simulink library "ConverterLibrary"  (R2026a)
settings: Solver=VariableStepAuto
undefined symbols (not defined in the file or in its folder): DiscIntNeverNeededParam, dspblkCoreblockFVToolHelper, gcbh, gridInverter
libraries: fl_lib x240, nesl_utility x221, ee_lib x208, slpidlib x28, eeGeneralControl x12, simulink x9, eeTransforms x4, simulink_extras x1, eePowerMeasurement x1
(part 11 of 30)

== system ConverterLibrary/Power Converter Plant/Soft-Switching Converters/LLC Converter/LLC Primary Inverter and Resonant Tank/LLC Simplified Model ==
  G : Inport
  Inverter : Subsystem
      settings: PortSchema="{\"entries\":[{\"content\":{\"sides\":[{\"content\":{\"connectorIds\":[\"LConn1\",\"LConn2\"]},\"type\":\"ConnectorPlacement.EquallySpacedRectSide\",\"uuid\":\"5f98eff0-54e4-47a8-aeeb-0279cba14f26\"},{\"content\":{\"connectorIds\":[\"RConn1\",\"RConn2\"],\"side\":\"RIGHT\"},\"type\":\"ConnectorPlacement.EquallySpacedRectSide\",\"uuid\":\"71acbbb6-1fc8-426c-b389-5d494eb18bfd\"},{\"content\":{\"connectorIds\":[\"In1\",\"Out1\"],\"side\":\"TOP\"},\"type\":\"ConnectorPlacement.EquallySpacedRectSide\",\"uuid\":\"dc77ee05-1f57-4323-bfda-b0076e2d1ee5\"}]},\"type\":\"ConnectorPlacement.EquallySpacedConnector\",\"uuid\":\"8d0b8c05-d5c5-4033-af60-ebdb639bdc40\"}],\"packageUris\":[\"http://schema.mathworks.com/mf0/Connector/R2020b\"],\"version\":\"1.0\"}"
  Resonant Tank : Subsystem
      settings: PortSchema="{\"entries\":[{\"content\":{\"sides\":[{\"content\":{\"connectorIds\":[\"LConn1\",\"LConn2\"]},\"type\":\"ConnectorPlacement.EquallySpacedRectSide\",\"uuid\":\"d505f362-3b8e-4dee-9b5b-731d75550efb\"},{\"content\":{\"connectorIds\":[\"RConn1\",\"RConn2\",\"RConn3\"],\"side\":\"RIGHT\"},\"type\":\"ConnectorPlacement.EquallySpacedRectSide\",\"uuid\":\"66ab4b84-9b7a-404b-b3f6-3ac1c371ea42\"},{\"content\":{\"connectorIds\":[\"Out1\"],\"side\":\"TOP\"},\"type\":\"ConnectorPlacement.EquallySpacedRectSide\",\"uuid\":\"00605859-d490-4a3b-aace-391362dfba7e\"}]},\"type\":\"ConnectorPlacement.EquallySpacedConnector\",\"uuid\":\"a210fe68-7181-499f-8e1c-ccfe71b42a4c\"}],\"packageUris\":[\"http://schema.mathworks.com/mf0/Connector/R2020b\"],\"version\":\"1.0\"}"
      mask Display: image('LLCTransformerIcon.png');
  Selector : Selector  InputPortWidth=4  IndexOptions=Index vector (dialog)  Indices=[1 2]  OutputSizes=1
  + : PMIOPort  Side=Left
  P2+ : PMIOPort  Port=2  Side=Right
  N2 : PMIOPort  Port=3  Side=Right
  - : PMIOPort  Port=4  Side=Left
  P2- : PMIOPort  Port=5  Side=Right
  measInv : Outport
  measTank : Outport  Port=2
  wires:
  Selector/1 -> Inverter/1(G)
  G/1 -> Selector/1
  Resonant Tank/1(meas) -> measTank/1  "ResonantTank"
  Inverter/1(meas) -> measInv/1  "Inverter"
  connections:
  Resonant Tank/RConn2 -- N2/RConn1
  +/RConn1 -- Inverter/LConn1
  Resonant Tank/RConn1 -- P2+/RConn1
  Resonant Tank/LConn2 -- Inverter/RConn2
  Resonant Tank/RConn3 -- P2-/RConn1
  Resonant Tank/LConn1 -- Inverter/RConn1
  -/RConn1 -- Inverter/LConn2

== system ConverterLibrary/Power Converter Plant/Soft-Switching Converters/LLC Converter/Rectifier/Iout ==
  Current Sensor : fl_lib/Electrical/Electrical Sensors/Current Sensor
  PS-Simulink Converter : nesl_utility/PS-Simulink Converter  PhysicalDomain=network_engine_domain  SubClassName=ps_output  LeftPortType=input  RightPortType=output  PseudoPeriodic=off  Frequencies=[]  VectorFormat=inherit  Unit=inherit  AffineConversion=off
  + : PMIOPort  Side=Left
  - : PMIOPort  Port=2  Side=Right
  I : Outport
  wires:
  PS-Simulink Converter/1 -> I/1
  connections:
  Current Sensor/RConn1 -- PS-Simulink Converter/LConn1
  +/RConn1 -- Current Sensor/LConn1
  Current Sensor/RConn2 -- -/RConn1

== system ConverterLibrary/Power Converter Plant/Soft-Switching Converters/LLC Converter/Rectifier/IoutRect ==
  Current Sensor : fl_lib/Electrical/Electrical Sensors/Current Sensor
  PS-Simulink Converter : nesl_utility/PS-Simulink Converter  PhysicalDomain=network_engine_domain  SubClassName=ps_output  LeftPortType=input  RightPortType=output  PseudoPeriodic=off  Frequencies=[]  VectorFormat=inherit  Unit=inherit  AffineConversion=off
  + : PMIOPort  Side=Left
  - : PMIOPort  Port=2  Side=Right
  I : Outport
  wires:
  PS-Simulink Converter/1 -> I/1
  connections:
  Current Sensor/RConn1 -- PS-Simulink Converter/LConn1
  +/RConn1 -- Current Sensor/LConn1
  Current Sensor/RConn2 -- -/RConn1

== system ConverterLibrary/Power Converter Plant/Soft-Switching Converters/LLC Converter/Rectifier/Rectifier Bridge ==
  Centre-Tap Ideal Diode : Subsystem  VariantControl=CentreTapIdealDiode
  Centre-Tap Tabulated Diode : Subsystem  VariantControl=CentreTapTabulatedDiode
  Full Bridge Ideal Diode : Subsystem  VariantControl=FullBridgeIdealDiode
  Full Bridge Tabulated Diode : Subsystem  VariantControl=FullBridgeTabulatedDiode
  P1+ : PMIOPort  Side=Left
  N1 : PMIOPort  Port=2  Side=Left
  P1- : PMIOPort  Port=3  Side=Left
  P2 : PMIOPort  Port=4  Side=Right
  N2 : PMIOPort  Port=5  Side=Right
  Ismeas : Outport

== system ConverterLibrary/Power Converter Plant/Soft-Switching Converters/LLC Converter/Rectifier/Subsystem4 ==
  PS-Simulink Converter : nesl_utility/PS-Simulink Converter  PhysicalDomain=network_engine_domain  SubClassName=ps_output  LeftPortType=input  RightPortType=output  PseudoPeriodic=off  Frequencies=[]  VectorFormat=inherit  Unit=inherit  AffineConversion=off
  Voltage Sensor : fl_lib/Electrical/Electrical Sensors/Voltage Sensor
  + : PMIOPort  Side=Left
  - : PMIOPort  Port=2  Side=Right
  V : Outport
  wires:
  PS-Simulink Converter/1 -> V/1
  connections:
  PS-Simulink Converter/LConn1 -- Voltage Sensor/RConn1
  Voltage Sensor/LConn1 -- +/RConn1
  Voltage Sensor/RConn2 -- -/RConn1

== system ConverterLibrary/Power Converter Plant/Soft-Switching Converters/LLC Converter/Rectifier/Vout ==
  PS-Simulink Converter : nesl_utility/PS-Simulink Converter  PhysicalDomain=network_engine_domain  SubClassName=ps_output  LeftPortType=input  RightPortType=output  PseudoPeriodic=off  Frequencies=[]  VectorFormat=inherit  Unit=inherit  AffineConversion=off
  Voltage Sensor : fl_lib/Electrical/Electrical Sensors/Voltage Sensor
  + : PMIOPort  Side=Left
  - : PMIOPort  Port=2  Side=Right
  V : Outport
  wires:
  PS-Simulink Converter/1 -> V/1
  connections:
  PS-Simulink Converter/LConn1 -- Voltage Sensor/RConn1
  Voltage Sensor/LConn1 -- +/RConn1
  Voltage Sensor/RConn2 -- -/RConn1

== system ConverterLibrary/Controller/Inverter-Based Resources/Grid-Forming Converter Controller/Current Limiting/CurrentLimitingMethod/currentLimitAndVirtual ==
  Igd : Inport
  Igq : Inport  Port=2
  Current Saturation : Subsystem
  CurrentLimitSelection : Stateflow chart  TreatAsAtomicUnit=on
  Math Function : Math  Operator=hypot
  Merge{,1..3} (4 alike) : Merge  Inputs=3
  No Fault Ride Through : Subsystem
  VI : Subsystem
  delVd : Outport
  delVq : Outport  Port=2
  Idmax : Outport  Port=3
  Iqmax : Outport  Port=4
  wires:
  [Imax] -> VI/3(Imax)
  [Imax] -> Current Saturation/3(Imaxsat)
  [noCtLt] -> No Fault Ride Through/Enable
  [satCtLt] -> Current Saturation/Enable
  [viCtLt] -> VI/Enable
  CurrentLimitSelection/4(satCurrentLimit) -> [satCtLt]
  CurrentLimitSelection/3(viCurrentLimit) -> [viCtLt]
  CurrentLimitSelection/2(noCurrentLimit) -> [noCtLt]
  CurrentLimitSelection/1(ismax) -> [Imax]
  Math Function/1 -> CurrentLimitSelection/1(Is)
  No Fault Ride Through/2(delVq) -> Merge1/3
  Merge3/1 -> Iqmax/1
  Current Saturation/2(delVq) -> Merge1/2
  No Fault Ride Through/4(iqmax) -> Merge3/3
  VI/3(idmax) -> Merge2/1
  VI/4(iqmax) -> Merge3/1
  Current Saturation/3(idmax) -> Merge2/2
  VI/2(delVq) -> Merge1/1
  Merge/1 -> delVd/1
  Current Saturation/4(iqmax) -> Merge3/2
  Current Saturation/1(delVd) -> Merge/2
  [Id] -> Math Function/1
  [Iq] -> Math Function/2
  VI/1(delVd) -> Merge/1
  No Fault Ride Through/3(idmax) -> Merge2/3
  No Fault Ride Through/1(delVd) -> Merge/3
  Igd/1 -> [Id], No Fault Ride Through/1(Id), Current Saturation/1(Id), VI/1(Id)
  Merge1/1 -> delVq/1
  Igq/1 -> [Iq], No Fault Ride Through/2(Iq), VI/2(Iq), Current Saturation/2(Iq)
  Merge2/1 -> Idmax/1

== system ConverterLibrary/Controller/Inverter-Based Resources/Grid-Forming Converter Controller/Current Limiting/CurrentLimitingMethod/currentSaturation ==
  note: Vs-delV
  Igd : Inport
  Igq : Inport  Port=2
  Compare : Subsystem
  Constant : Constant  Value=maxSatCurrentLimit
  Constant1 : Constant  Value=0
  Constant2 : Constant  Value=0
  If : If
  If Action Subsystem : Subsystem  TreatAsAtomicUnit=on
  If Action Subsystem1 : Subsystem  TreatAsAtomicUnit=on
  Math Function : Math  Operator=hypot
  Merge : Merge
  Merge1 : Merge
  Subtract : Sum  Inputs=-+
  delVd : Outport
  delVq : Outport  Port=2
  Idmax : Outport  Port=3
  Iqmax : Outport  Port=4
  wires:
  Merge1/1 -> Iqmax/1
  Merge/1 -> Idmax/1
  Constant1/1 -> delVd/1
  Constant2/1 -> delVq/1
  If Action Subsystem1/2(Iqmax) -> Merge1/2
  If Action Subsystem/2(Iqmax) -> Merge1/1
  If Action Subsystem1/1(Idmax) -> Merge/2
  If Action Subsystem/1(Idmax) -> Merge/1
  [Is] -> If Action Subsystem/1(Is)
  If/2 -> If Action Subsystem1/Action
  Compare/1(Out1) -> If/1
  Subtract/1 -> Compare/1(u)
  [Isq] -> If Action Subsystem/3(Isq)
  [Isd] -> If Action Subsystem/2(Isd)
  If/1 -> If Action Subsystem/Action
  Math Function/1 -> Subtract/2, [Is]  "Is"
  Constant/1 -> Subtract/1
  Igq/1 -> Math Function/2, [Isq]
  Igd/1 -> Math Function/1, [Isd]

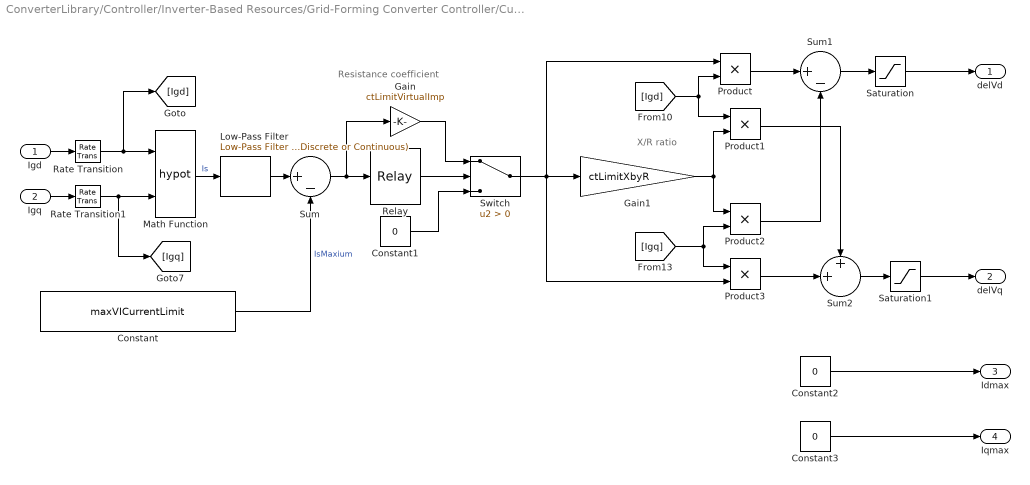
== system ConverterLibrary/Controller/Inverter-Based Resources/Grid-Forming Converter Controller/Current Limiting/CurrentLimitingMethod/virtualImpedance ==
  note: Resistance coefficient
  note: X/R ratio
  Igd : Inport
  Igq : Inport  Port=2
  Constant : Constant  Value=maxVICurrentLimit
  Constant1 : Constant  Value=0
  Constant2 : Constant  Value=0
  Constant3 : Constant  Value=0
  Gain : Gain  Gain=ctLimitVirtualImp
  Gain1 : Gain  Gain=ctLimitXbyR
  Low-Pass Filter : eeGeneralControl/Low-Pass Filter (Discrete or Continuous)  K=1  T=currentVITimeConst  B=inf  A=-inf  init_option=Inherited from block input  x0=0  Ts=-1
  Math Function : Math  Operator=hypot
  Product{,1..3} (4 alike) : Product
  Rate Transition : RateTransition
  Rate Transition1 : RateTransition
  Relay : Relay  OnSwitchValue=0.01  OffSwitchValue=-0.05
  Saturation : Saturate  UpperLimit=1  LowerLimit=-1
  Saturation1 : Saturate  UpperLimit=1  LowerLimit=-1
  Sum : Sum  Inputs=|+-
  Sum1 : Sum  Inputs=|+-
  Sum2 : Sum  Inputs=++|
  Switch : Switch  Criteria=u2 > Threshold  SaturateOnIntegerOverflow=off  InputSameDT=off
  delVd : Outport
  delVq : Outport  Port=2
  Idmax : Outport  Port=3
  Iqmax : Outport  Port=4
  wires:
  Rate Transition1/1 -> Math Function/2, [Igq]
  Rate Transition/1 -> [Igd], Math Function/1
  Sum2/1 -> Saturation1/1
  Product3/1 -> Sum2/2
  Low-Pass Filter/1 -> Sum/1
  Saturation/1 -> delVd/1
  Relay/1 -> Switch/2
  Saturation1/1 -> delVq/1
  Igd/1 -> Rate Transition/1
  Constant1/1 -> Switch/3
  Gain/1 -> Switch/1
  Constant3/1 -> Iqmax/1
  Constant2/1 -> Idmax/1
  [Igd] -> Product/2, Product1/1
  Switch/1 -> Product/1, Product3/2, Gain1/1
  [Igq] -> Product2/2, Product3/1
  Math Function/1 -> Low-Pass Filter/1  "Is"
  Constant/1 -> Sum/2  "IsMaxium"
  Product2/1 -> Sum1/2
  Product/1 -> Sum1/1
  Sum1/1 -> Saturation/1
  Gain1/1 -> Product2/1, Product1/2
  Product1/1 -> Sum2/1
  Igq/1 -> Rate Transition1/1
  Sum/1 -> Relay/1, Gain/1

== system ConverterLibrary/Controller/Inverter-Based Resources/Grid-Forming Converter Controller/Grid Voltage Reactive Power Support/Modifying Active Power Reference/Computing New Active Power Ref ==
  Iq : Inport
  Vd : Inport  Port=2
  Abs : Abs  SaturateOnIntegerOverflow=off
  Constant : Constant  Value=maxVICurrentLimit*0.96
  Constant1 : Constant  Value=0
  Product : Product
  Sqrt : Sqrt
  Square : Math  Operator=square
  Square1 : Math  Operator=square
  Subtract : Sum  Inputs=-+
  Switch : Switch  Criteria=u2 > Threshold  Threshold=1.15  SaturateOnIntegerOverflow=off  InputSameDT=off
  Pref : Outport
  wires:
  Abs/1 -> Switch/1
  Constant1/1 -> Switch/3
  Subtract/1 -> Sqrt/1, Switch/2
  Product/1 -> Pref/1
  Iq/1 -> Square/1
  Sqrt/1 -> Abs/1
  Vd/1 -> Product/1
  Square1/1 -> Subtract/2
  Square/1 -> Subtract/1
  Switch/1 -> Product/2
  Constant/1 -> Square1/1

== system ConverterLibrary/Controller/Inverter-Based Resources/Grid-Forming Converter Controller/Grid Voltage Reactive Power Support/Modifying Reactive Power Reference/Changing the Power Reference ==
  Vs : Inport
  Vd : Inport  Port=2
  Pref : Inport  Port=3
  Qref : Inport  Port=4
  Enable : EnablePort
  ActivePowerReference : Subsystem
  Constant1 : Constant  Value=voltreference*0.96
  Estimate Id for Given Iq : Subsystem
  EstimateIqForReactivePower : Subsystem
  Max : MinMax  Function=max  Inputs=2
  ReactivePowerReference : Subsystem
  Prefv : Outport
  Qrefv : Outport  Port=2
  wires:
  Vd/1 -> EstimateIqForReactivePower/2(Vd)
  Qref/1 -> Max/2
  Max/1 -> Qrefv/1
  ReactivePowerReference/1(QrefNew) -> Max/1
  ActivePowerReference/1(PrefNew) -> Prefv/1
  Pref/1 -> ActivePowerReference/3(Pref)
  Estimate Id for Given Iq/1(Id) -> ActivePowerReference/1(Id)
  Vs/1 -> ReactivePowerReference/1(Vd), EstimateIqForReactivePower/3(Vs), ActivePowerReference/2(Vd)
  Constant1/1 -> EstimateIqForReactivePower/1(Vmin)
  EstimateIqForReactivePower/1(Iq) -> ReactivePowerReference/2(Iq), Estimate Id for Given Iq/1(Iq)

== system ConverterLibrary/Controller/Inverter-Based Resources/Grid-Forming Converter Controller/Grid Voltage Reactive Power Support/Modifying Reactive Power Reference/Hysteresis ==
  Vs : Inport
  AND : Logic  IconShape=distinctive  AllPortsSameDT=off  OutDataTypeStr=boolean
  Compare To Constant : simulink/Logic and Bit Operations/Compare To Constant  relop=<  const=0.9  OutDataTypeStr=boolean
  Compare To Constant1 : simulink/Logic and Bit Operations/Compare To Constant  relop=<  const=0.95  OutDataTypeStr=boolean
  D Latch : simulink_extras/Flip Flops/D Latch
  OR : Logic  Operator=OR  IconShape=distinctive  AllPortsSameDT=off  OutDataTypeStr=boolean
  Terminator : Terminator
  LVFlag : Outport
  wires:
  Vs/1 -> Compare To Constant/1, Compare To Constant1/1
  Compare To Constant/1 -> OR/2, D Latch/2, D Latch/1
  D Latch/2 -> Terminator/1
  OR/1 -> LVFlag/1
  AND/1 -> OR/1
  D Latch/1 -> AND/2
  Compare To Constant1/1 -> AND/1

== system ConverterLibrary/Controller/Inverter-Based Resources/Grid-Forming Converter Controller/Grid Voltage Reactive Power Support/Modifying Reactive Power Reference/Not Altering the Power Reference ==
  Pref : Inport
  Qref : Inport  Port=2
  Enable : EnablePort
  Prefv : Outport
  Qrefv : Outport  Port=2
  wires:
  Qref/1 -> Qrefv/1
  Pref/1 -> Prefv/1

== system ConverterLibrary/Controller/Inverter-Based Resources/Grid-Forming Converter Controller/Measurement/Frequency Measurement/Frequency Measurement ==
  abc : Inport
  Constant : Constant
  Discrete-Time Integrator : DiscreteIntegrator  SampleTime=sampleTime  LimitOutput=on  ICPrevOutput=DiscIntNeverNeededParam  ICPrevScaledInput=DiscIntNeverNeededParam
  If : If  IfExpression=u1 > 0.9
  If Action Subsystem : Subsystem  TreatAsAtomicUnit=on
  If Action Subsystem1 : Subsystem  TreatAsAtomicUnit=on
  Merge : Merge
  Postive Sequence : Subsystem
  Freq : Outport
  wires:
  Postive Sequence/1(posSeq) -> If Action Subsystem/1(V)
  Merge/1 -> Freq/1
  If Action Subsystem1/1(Out1) -> Merge/2
  If Action Subsystem/1(Freq) -> Merge/1
  Constant/1 -> Discrete-Time Integrator/1
  abc/1 -> Postive Sequence/1(abc)
  Discrete-Time Integrator/1 -> If/1, If Action Subsystem/2(Time)
  If/2 -> If Action Subsystem1/Action
  If/1 -> If Action Subsystem/Action

== system ConverterLibrary/Controller/Inverter-Based Resources/Grid-Forming Converter Controller/Measurement/abc2dq/Supply Current to dq ==
  abc : Inport
  Angle : Inport  Port=2
  Demux : Demux  Outputs=3
  Park Transform : eeTransforms/Park Transform  AxisAlignment=D-axis  PowerInvariant=off
  Terminator : Terminator
  Igd : Outport  VectorParamsAs1DForOutWhenUnconnected=off
  Igq : Outport  Port=2  VectorParamsAs1DForOutWhenUnconnected=off
  wires:
  Angle/1 -> Park Transform/2
  abc/1 -> Park Transform/1
  Demux/1 -> Igd/1
  Demux/2 -> Igq/1
  Park Transform/1 -> Demux/1
  Demux/3 -> Terminator/1

== system ConverterLibrary/Controller/Inverter-Based Resources/Grid-Forming Converter Controller/Measurement/abc2dq/Supply Voltage  to dq ==
  Angle : Inport
  abc : Inport  Port=2
  Demux : Demux  Outputs=3
  Park Transform : eeTransforms/Park Transform  AxisAlignment=D-axis  PowerInvariant=off
  Terminator : Terminator
  Vgd : Outport  VectorParamsAs1DForOutWhenUnconnected=off
  Vgq : Outport  Port=2  VectorParamsAs1DForOutWhenUnconnected=off
  wires:
  Angle/1 -> Park Transform/2
  abc/1 -> Park Transform/1
  Demux/1 -> Vgd/1
  Demux/2 -> Vgq/1
  Park Transform/1 -> Demux/1
  Demux/3 -> Terminator/1

== system ConverterLibrary/Controller/Inverter-Based Resources/Grid-Forming Converter Controller/Power Control/ActivePowerControl/droopControl ==
  Pref : Inport
  Pmeas : Inport  Port=2
  fgrid : Inport  Port=3
  Add : Sum  Inputs=+-
  Constant : Constant
  Constant5 : Constant  Value=pi/2
  Gain : Gain  Gain=powerFreq*2*pi
  Integrator with Wrapped State (Discrete or Continuous) : eeGeneralControl/Integrator with Wrapped State (Discrete or Continuous)  LabelModeActiveChoice=Discrete  WrappedStateUpperValue=2*pi  WrappedStateLowerValue=0  x0=0  Ts=activePowerSampleTime
      settings: LibrarySourceBlock=|
      | ee_sl_lib/General Control/Integrator with
      | Wrapped State
      | (Discrete or Continuous)
  Lead-Lag (Discrete or Continuous) : eeGeneralControl/Lead-Lag (Discrete or Continuous)  T1=droopT1  T2=droopT2  B=inf  A=-inf  init_option=Inherited from block input  x0=0  Ts=activePowerSampleTime
      settings: LibrarySourceBlock=|
      | ee_sl_lib/General Control/Lead-Lag
      | (Discrete or Continuous)
  Low-Pass Filter (Discrete or Continuous) : eeGeneralControl/Low-Pass Filter (Discrete or Continuous)  K=1  T=droopTC  B=inf  A=-inf  init_option=Specify as parameter  x0=0  Ts=activePowerSampleTime
  Sum : Sum  Inputs=|-+
  Sum1 : Sum  Inputs=|-+
  Terminator : Terminator
  mp : Gain  Gain=droopSlope
  Theta : Outport
  w : Outport  Port=2
  wires:
  fgrid/1 -> Terminator/1
  Sum1/1 -> Gain/1
  Constant/1 -> Sum1/2
  Integrator with Wrapped State (Discrete or Continuous)/1 -> Add/1
  Lead-Lag (Discrete or Continuous)/1 -> Sum/2
  Gain/1 -> w/1, Integrator with Wrapped State (Discrete or Continuous)/1
  Pref/1 -> Sum/1
  Constant5/1 -> Add/2
  Add/1 -> Theta/1
  Pmeas/1 -> Lead-Lag (Discrete or Continuous)/1
  Sum/1 -> mp/1
  mp/1 -> Low-Pass Filter (Discrete or Continuous)/1
  Low-Pass Filter (Discrete or Continuous)/1 -> Sum1/1

== system ConverterLibrary/Controller/Inverter-Based Resources/Grid-Forming Converter Controller/Power Control/ActivePowerControl/vsmControl ==
  note: Damping power input
  note: Frequency difference power
  note: Measured power
  Pref : Inport
  Pmeas : Inport  Port=2
  fgrid : Inport  Port=3
  Add : Sum  Inputs=+-
  Constant : Constant
  Constant2 : Constant  Value=pi/2
  Damping Frequency : Subsystem  Variant=on  VariantControlMode=label  VariantControl=Choice  LabelModeActiveChoice=freqMeas
  Discrete-Time Integrator : DiscreteIntegrator  IntegratorMethod=Integration: Backward Euler  InitialCondition=1  SampleTime=activePowerSampleTime  LimitOutput=on  UpperSaturationLimit=1.1  LowerSaturationLimit=0.9  ICPrevOutput=DiscIntNeverNeededParam  ICPrevScaledInput=DiscIntNeverNeededParam
  Gain : Gain  Gain=powerFreq*2*pi
  Gain1 : Gain  Gain=1/vsmInertiaTC
  Gain2 : Gain  Gain=vsmDampingConst*powerFreq
  Gain6 : Gain  Gain=vsmFreqDroop
  Integrator with Wrapped State (Discrete or Continuous) : eeGeneralControl/Integrator with Wrapped State (Discrete or Continuous)  LabelModeActiveChoice=Discrete  WrappedStateUpperValue=2*pi  WrappedStateLowerValue=0  x0=0  Ts=activePowerSampleTime
      settings: LibrarySourceBlock=|
      | ee_sl_lib/General Control/Integrator with
      | Wrapped State
      | (Discrete or Continuous)
  Low-Pass Filter (Discrete or Continuous) : eeGeneralControl/Low-Pass Filter (Discrete or Continuous)  K=1  T=vsmPmeasFilterTC  B=inf  A=-inf  init_option=Specify as parameter  x0=0  Ts=activePowerSampleTime
  Saturation : Saturate  UpperLimit=dampingPowerMaxLimit  LowerLimit=dampingPowerMinLimit
  Sum : Sum  Inputs=|+-
  Sum1 : Sum  Inputs=-+-|
  Sum2 : Sum  Inputs=|+-
  Sum3 : Sum  Inputs=++|
  Unit Delay : UnitDelay  SampleTime=-1
  Unit Delay1 : UnitDelay  SampleTime=-1
  Theta : Outport
  w : Outport  Port=2
  wires:
  Damping Frequency/1(fmeas) -> Sum2/2
  fgrid/1 -> Damping Frequency/1(fref)
  Gain6/1 -> Sum3/2
  Saturation/1 -> Sum1/3  "Pdamping"
  Unit Delay1/1 -> [Wsm]
  Constant/1 -> Sum/1
  Unit Delay/1 -> Gain2/1
  Gain/1 -> w/1, Integrator with Wrapped State (Discrete or Continuous)/1
  Gain1/1 -> Discrete-Time Integrator/1
  Sum2/1 -> Unit Delay/1
  Sum3/1 -> Sum1/2
  Gain2/1 -> Saturation/1
  Pref/1 -> Sum3/1  "Reference power"
  Low-Pass Filter (Discrete or Continuous)/1 -> Sum1/1
  [Wsm] -> Sum/2
  Discrete-Time Integrator/1 -> Sum2/1, Unit Delay1/1, Gain/1
  Pmeas/1 -> Low-Pass Filter (Discrete or Continuous)/1
  Add/1 -> Theta/1
  Constant2/1 -> Add/2
  Sum/1 -> Gain6/1
  Sum1/1 -> Gain1/1  "Pinertia"
  Integrator with Wrapped State (Discrete or Continuous)/1 -> Add/1

== system ConverterLibrary/Controller/Inverter-Based Resources/Grid-Forming Converter Controller/VoltageCurrentControl/Controller/Id Current Limiting ==
  Imax : Inport
  Id : Inport  Port=2
  Abs : Abs  SaturateOnIntegerOverflow=off
  Rate Transition : RateTransition
  Switch : Switch  Criteria=u2 > Threshold  SaturateOnIntegerOverflow=off  InputSameDT=off
  Idref : Outport
  wires:
  Rate Transition/1 -> Switch/3
  Switch/1 -> Idref/1
  Imax/1 -> Switch/1, Abs/1
  Abs/1 -> Switch/2
  Id/1 -> Rate Transition/1

== system ConverterLibrary/Controller/Inverter-Based Resources/Grid-Forming Converter Controller/VoltageCurrentControl/Controller/Iq Current Limiting ==
  Imax : Inport
  Iq : Inport  Port=2
  Abs : Abs  SaturateOnIntegerOverflow=off
  Switch : Switch  Criteria=u2 > Threshold  SaturateOnIntegerOverflow=off  InputSameDT=off
  Iqref : Outport
  wires:
  Switch/1 -> Iqref/1
  Imax/1 -> Switch/1, Abs/1
  Abs/1 -> Switch/2
  Iq/1 -> Switch/3

== system ConverterLibrary/Controller/Inverter-Based Resources/Grid-Forming Converter Controller/VoltageCurrentControl/Controller/Voltage control ==
  e : Inport
  Discrete-Time Integrator : DiscreteIntegrator  IntegratorMethod=Integration: Backward Euler  SampleTime=voltControlTs  LimitOutput=on  UpperSaturationLimit=VdMaxCt  LowerSaturationLimit=VdMinCt  ICPrevOutput=DiscIntNeverNeededParam  ICPrevScaledInput=DiscIntNeverNeededParam
  Ki : Gain  Gain=VdIGain
  Kp : Gain  Gain=vdPGain
  Limit : Saturate  UpperLimit=VdMaxCt  LowerLimit=VdMinCt
  Sum7 : Sum  Inputs=|++
  u : Outport  VectorParamsAs1DForOutWhenUnconnected=off
  wires:
  e/1 -> Ki/1, Kp/1
  Sum7/1 -> Limit/1
  Ki/1 -> Discrete-Time Integrator/1
  Limit/1 -> u/1
  Kp/1 -> Sum7/1
  Discrete-Time Integrator/1 -> Sum7/2

== system ConverterLibrary/Controller/Inverter-Based Resources/Grid-Forming Converter Controller/VoltageCurrentControl/Controller/Voltage control1 ==
  e : Inport
  Discrete-Time Integrator : DiscreteIntegrator  IntegratorMethod=Integration: Backward Euler  SampleTime=voltControlTs  LimitOutput=on  UpperSaturationLimit=VqMaxCt  LowerSaturationLimit=VqMinCt  ICPrevOutput=DiscIntNeverNeededParam  ICPrevScaledInput=DiscIntNeverNeededParam
  Ki : Gain  Gain=VqIGain
  Kp : Gain  Gain=VqPGain
  Limit : Saturate  UpperLimit=VqMaxCt  LowerLimit=VqMinCt
  Sum7 : Sum  Inputs=|++
  u : Outport  VectorParamsAs1DForOutWhenUnconnected=off
  wires:
  Limit/1 -> u/1
  Ki/1 -> Discrete-Time Integrator/1
  Kp/1 -> Sum7/1
  e/1 -> Kp/1, Ki/1
  Sum7/1 -> Limit/1
  Discrete-Time Integrator/1 -> Sum7/2

== system ConverterLibrary/Controller/Inverter-Based Resources/Grid-Forming Converter Controller/VoltageCurrentControl/Controller/d-axis current control ==
  e : Inport
  Discrete-Time Integrator : DiscreteIntegrator  IntegratorMethod=Integration: Backward Euler  SampleTime=currentControlTs  LimitOutput=on  UpperSaturationLimit=4  LowerSaturationLimit=-4  ICPrevOutput=DiscIntNeverNeededParam  ICPrevScaledInput=DiscIntNeverNeededParam
  Ki : Gain  Gain=IdIGain
  Kp : Gain  Gain=IdPGain
  Limit : Saturate  UpperLimit=4  LowerLimit=-4
  Sum7 : Sum  Inputs=|++
  u : Outport  VectorParamsAs1DForOutWhenUnconnected=off
  wires:
  Ki/1 -> Discrete-Time Integrator/1
  Limit/1 -> u/1
  Kp/1 -> Sum7/1
  e/1 -> Kp/1, Ki/1
  Sum7/1 -> Limit/1
  Discrete-Time Integrator/1 -> Sum7/2

== system ConverterLibrary/Controller/Inverter-Based Resources/Grid-Forming Converter Controller/VoltageCurrentControl/Controller/q-axis current control ==
  e : Inport
  Discrete-Time Integrator : DiscreteIntegrator  IntegratorMethod=Integration: Backward Euler  SampleTime=currentControlTs  LimitOutput=on  UpperSaturationLimit=3  LowerSaturationLimit=-3  ICPrevOutput=DiscIntNeverNeededParam  ICPrevScaledInput=DiscIntNeverNeededParam
  Ki : Gain  Gain=IqIGain
  Kp : Gain  Gain=IqPGain
  Limit : Saturate  UpperLimit=3  LowerLimit=-3
  Sum7 : Sum  Inputs=|++
  u : Outport  VectorParamsAs1DForOutWhenUnconnected=off
  wires:
  Discrete-Time Integrator/1 -> Sum7/2
  Limit/1 -> u/1
  Sum7/1 -> Limit/1
  e/1 -> Ki/1, Kp/1
  Kp/1 -> Sum7/1
  Ki/1 -> Discrete-Time Integrator/1

== system ConverterLibrary/Controller/Non-Isolated DC-DC Converters/Non-Isolated DC-DC Controller/Duty Feedforward/Feedforward Law/Boost ==
  voltageReferencePu : Inport
  inputVoltagePuOut : Inport  Port=2
  Feedforward One : Constant
  Sum : Sum  Inputs=|+-
  Voltage Ratio : Product  Inputs=*/
  dutyFeedforward : Outport
  wires:
  Sum/1 -> dutyFeedforward/1
  Voltage Ratio/1 -> Sum/2
  Feedforward One/1 -> Sum/1
  voltageReferencePu/1 -> Voltage Ratio/2
  inputVoltagePuOut/1 -> Voltage Ratio/1

== system ConverterLibrary/Controller/Non-Isolated DC-DC Converters/Non-Isolated DC-DC Controller/Duty Feedforward/Feedforward Law/Buck ==
  voltageReferencePu : Inport
  inputVoltagePuOut : Inport  Port=2
  Voltage Ratio : Product  Inputs=*/
  dutyFeedforward : Outport
  wires:
  Voltage Ratio/1 -> dutyFeedforward/1
  inputVoltagePuOut/1 -> Voltage Ratio/2
  voltageReferencePu/1 -> Voltage Ratio/1

== system ConverterLibrary/Controller/Non-Isolated DC-DC Converters/Non-Isolated DC-DC Controller/Duty Feedforward/Feedforward Law/BuckBoost ==
  voltageReferencePu : Inport
  inputVoltagePuOut : Inport  Port=2
  Sum : Sum  Inputs=|++
  Voltage Ratio : Product  Inputs=*/
  dutyFeedforward : Outport
  wires:
  Voltage Ratio/1 -> dutyFeedforward/1
  inputVoltagePuOut/1 -> Sum/2
  voltageReferencePu/1 -> Voltage Ratio/1, Sum/1
  Sum/1 -> Voltage Ratio/2

== system ConverterLibrary/Controller/Non-Isolated DC-DC Converters/Non-Isolated DC-DC Controller/Loop Structure/DoubleLoop/Current Controller ==
  error : Inport
  up : Inport  Port=2
  lo : Inport  Port=3
  PIContinuous : Subsystem  VariantControl=PIContinuous
  PIDiscrete : Subsystem  VariantControl=PIDiscrete
  vc : Outport

== system ConverterLibrary/Controller/Non-Isolated DC-DC Converters/Non-Isolated DC-DC Controller/Output Mode/PWMSignal/Half Bridge PWM Generator ==
  duty : Inport
  Dead Time : Constant  Value=(pwmDeadTime)
  Gate Level Offset : Bias  Bias=gateVoltageOff
  Gate Level Swing : Gain  Gain=gateVoltageOn - gateVoltageOff
  Leg Gate Logic : Subsystem
  Pulse Time : Gain  Gain=1/Fsw
  Pulse Time Plus Dead Time : Bias  Bias=(pwmDeadTime)
  Pulse Width Limit : Saturate  UpperLimit=1 - (pwmDeadTime)*Fsw  LowerLimit=(pwmDeadTime)*Fsw
  Ramp Mode : Subsystem  Variant=on  VariantControlMode=label  LabelModeActiveChoice=VariableStep
  Switching Period : Constant  Value=1/Fsw
  Turn Off Times : Mux  Inputs=2
  Turn On Times : Mux  Inputs=2
  G : Outport
  wires:
  duty/1 -> Pulse Width Limit/1
  Pulse Width Limit/1 -> Pulse Time/1
  Pulse Time/1 -> Pulse Time Plus Dead Time/1, Turn Off Times/1
  Dead Time/1 -> Turn On Times/1
  Pulse Time Plus Dead Time/1 -> Turn On Times/2
  Switching Period/1 -> Turn Off Times/2, Ramp Mode/1(Tsw)
  Gate Level Swing/1 -> Gate Level Offset/1
  Turn On Times/1 -> Leg Gate Logic/1(Ton)
  Turn Off Times/1 -> Leg Gate Logic/2(Toff)
  Ramp Mode/1(S) -> Leg Gate Logic/3(S)
  Leg Gate Logic/1(gates) -> Gate Level Swing/1
  Gate Level Offset/1 -> G/1

== system ConverterLibrary/Controller/PWM Generators/CLLC PWM Generator/Primary Gate Signal/Ramp Mode/FixedStep ==
  Tsw : Inport
  Initial Ramp Value : InitialCondition  Value=0
  Overshoot Residual : Sum  Inputs=-+
  Period Reached : RelationalOperator  Operator=>  ZeroCross=off
  Time Ramp : DiscreteIntegrator  ExternalReset=rising  InitialConditionSource=external  SampleTime=Ts  ShowStatePort=on  ICPrevOutput=DiscIntNeverNeededParam  ICPrevScaledInput=DiscIntNeverNeededParam
  Unit Rate : Constant
  S : Outport
  wires:
  Unit Rate/1 -> Time Ramp/1
  Period Reached/1 -> Time Ramp/2
  Time Ramp/1 -> S/1
  Tsw/1 -> Overshoot Residual/1, Period Reached/2
  Time Ramp/State -> Period Reached/1, Overshoot Residual/2
  Overshoot Residual/1 -> Initial Ramp Value/1
  Initial Ramp Value/1 -> Time Ramp/3

== system ConverterLibrary/Controller/PWM Generators/CLLC PWM Generator/Primary Gate Signal/Ramp Mode/VariableStep ==
  Tsw : Inport
  Initial Ramp Value : InitialCondition  Value=0
  Overshoot Residual : Sum  Inputs=-+
  Period Reached : RelationalOperator  Operator=>
  Time Ramp : Integrator  ExternalReset=rising  InitialConditionSource=external  ShowStatePort=on
  Unit Rate : Constant
  S : Outport
  wires:
  Unit Rate/1 -> Time Ramp/1
  Period Reached/1 -> Time Ramp/2
  Time Ramp/1 -> S/1
  Tsw/1 -> Overshoot Residual/1, Period Reached/2
  Time Ramp/State -> Period Reached/1, Overshoot Residual/2
  Overshoot Residual/1 -> Initial Ramp Value/1
  Initial Ramp Value/1 -> Time Ramp/3

== system ConverterLibrary/Controller/PWM Generators/CLLC PWM Generator/Synchronous Rectifier/Region Select/Above Resonance ==
  primaryGates : Inport
  permit : Inport  Port=2
  Action Port : ActionPort
  Unused Primary Gates : Terminator
  Gs : Outport  InitialOutput=0
  wires:
  primaryGates/1 -> Unused Primary Gates/1
  permit/1 -> Gs/1

== system ConverterLibrary/Controller/PWM Generators/CLLC PWM Generator/Synchronous Rectifier/Region Select/Below Resonance ==
  primaryGates : Inport
  permit : Inport  Port=2
  Action Port : ActionPort
  Rectifier Permit : Logic
  Gs : Outport  InitialOutput=0
  wires:
  primaryGates/1 -> Rectifier Permit/1
  permit/1 -> Rectifier Permit/2
  Rectifier Permit/1 -> Gs/1

== system ConverterLibrary/Controller/PWM Generators/CLLC PWM Generator/Synchronous Rectifier/Region Select/Within Band ==
  primaryGates : Inport
  permit : Inport  Port=2
  Action Port : ActionPort
  Unused Rectifier Permit : Terminator
  Gs : Outport  InitialOutput=0
  wires:
  permit/1 -> Unused Rectifier Permit/1
  primaryGates/1 -> Gs/1

== system ConverterLibrary/Controller/PWM Generators/CLLC PWM Generator/Synchronous Rectifier/Turn On Delay/Rectifier Ramp Mode ==
  rate : Inport
  FixedStep : Subsystem  VariantControl=FixedStep
  VariableStep : Subsystem  VariantControl=VariableStep
  S : Outport

== system ConverterLibrary/Controller/Power Factor Correction Converters/Boost PFC Controller/Output Mode/PWMSignal/Gate Drive ==
  gateLogic : Inport
  Gate Level Span : Gain  Gain=gateVoltageOn - gateVoltageOff
  Gate Off Level : Bias  Bias=gateVoltageOff  SaturateOnIntegerOverflow=off
  gateVoltage : Outport
  wires:
  Gate Off Level/1 -> gateVoltage/1
  Gate Level Span/1 -> Gate Off Level/1
  gateLogic/1 -> Gate Level Span/1

== system ConverterLibrary/Controller/Power Factor Correction Converters/Boost PFC Controller/Output Mode/PWMSignal/Leg Gate Logic ==
  Ton : Inport
  Toff : Inport  Port=2
  S : Inport  Port=3
  After Turn Off : RelationalOperator
  After Turn On : RelationalOperator
  Pulse Window : Logic  Operator=XOR
  To Double : DataTypeConversion  OutDataTypeStr=double
  gates : Outport
  wires:
  Ton/1 -> After Turn On/2
  Toff/1 -> After Turn Off/2
  S/1 -> After Turn Off/1, After Turn On/1
  After Turn On/1 -> Pulse Window/1
  After Turn Off/1 -> Pulse Window/2
  Pulse Window/1 -> To Double/1
  To Double/1 -> gates/1

== system ConverterLibrary/Controller/Power Factor Correction Converters/Boost PFC Controller/Output Mode/PWMSignal/Ramp Mode ==
  Tsw : Inport
  FixedStep : Subsystem  VariantControl=FixedStep
  VariableStep : Subsystem  VariantControl=VariableStep
  S : Outport

== system ConverterLibrary/Controller/Power Factor Correction Converters/Interleaved Boost PFC Controller/Current Balance/Balance Controller/PIContinuous ==
  error : Inport
  PI Controller : slpidlib/PID Controller  Controller=PI  Form=Parallel  TimeDomain=Continuous-time  UseExternalTs=off  SampleTime=-1  IntegratorMethod=Forward Euler  FilterMethod=Forward Euler  ControllerParametersSource=internal  P=KpBalance  I=KiBalance  UseKiTs=off  D=0  UseExternalDerivativeSource=off  N=100  UseFilter=on  TunerSelectOption=Transfer Function Based (PID Tuner App)  InitialConditionSource=internal  InitialConditionForIntegrator=0  InitialConditionForFilter=0  DifferentiatorICPrevScaledInput=0  ExternalReset=none  TrackingMode=off  Kt=1  LimitOutput=on  SatLimitsSource=internal  UpperSaturationLimit=dutyBalanceMax  LowerSaturationLimit=-dutyBalanceMax  LinearizeAsGain=on  AntiWindupMode=clamping  Kb=1  LimitIntegrator=on  UpperIntegratorSaturationLimit=dutyBalanceMax  LowerIntegratorSaturationLimit=-dutyBalanceMax  POutMin=[]  POutMax=[]  IOutMin=[]  IOutMax=[]  DOutMin=[]  DOutMax=[]  NOutMin=[]  NOutMax=[]  SumOutMin=[]  SumOutMax=[]  SaturationOutMin=[]  SaturationOutMax=[]  PParamMin=[]  PParamMax=[]  IParamMin=[]  IParamMax=[]  DParamMin=[]  DParamMax=[]  NParamMin=[]  NParamMax=[]  KbParamMin=[]  KbParamMax=[]  KtParamMin=[]  KtParamMax=[]  KbOutMin=[]  KbOutMax=[]  KtOutMin=[]  KtOutMax=[]  IntegratorOutMin=[]  IntegratorOutMax=[]  FilterOutMin=[]  FilterOutMax=[]  SumI1OutMin=[]  SumI1OutMax=[]  SumI2OutMin=[]  SumI2OutMax=[]  SumI3OutMin=[]  SumI3OutMax=[]  SumI4OutMin=[]  SumI4OutMax=[]  SumDOutMin=[]  SumDOutMax=[]  DifferentiatorOutMin=[]  DifferentiatorOutMax=[]  FilterDiffOutCoefMin=[]  FilterDiffOutCoefMax=[]  ReciprocalOutMin=[]  ReciprocalOutMax=[]  SumDenOutMin=[]  SumDenOutMax=[]  SumNumOutMin=[]  SumNumOutMax=[]  DivideOutMin=[]  DivideOutMax=[]  UdiffTsProdOutMin=[]  UdiffTsProdOutMax=[]  NTsProdOutMin=[]  NTsProdOutMax=[]  UintegralTsProdOutMin=[]  UintegralTsProdOutMax=[]  UngainTsProdOutMin=[]  UngainTsProdOutMax=[]  ClampingZeroOutDataTypeStr=Inherit: Inherit via back propagation  ClampingZeroOutMin=[]  ClampingZeroOutMax=[]  FilterDenConstantOutDataTypeStr=Inherit: Inherit via back propagation  FilterDenConstantOutMin=[]  FilterDenConstantOutMax=[]  PCopyOutDataTypeStr=Inherit: Inherit via back propagation  PCopyOutMin=[]  PCopyOutMax=[]  NCopyOutDataTypeStr=Inherit: Inherit via back propagation  NCopyOutMin=[]  NCopyOutMax=[]  IntegratorContinuousStateAttributes=''  IntegratorStateMustResolveToSignalObject=off  IntegratorRTWStateStorageClass=Auto  FilterContinuousStateAttributes=''  FilterStateMustResolveToSignalObject=off  FilterRTWStateStorageClass=Auto  ParallelPVariant=InternalParameters  IdealPVariant=Disabled  IVariant=InternalParameters  DVariant=Disabled  IntegratorVariant=Continuous  SatVariant=Enabled  AWVariant=ContClampingParallel  PCopyVariant=Disabled  TRVariant=Disabled  FdbkBlocksVariant=Forward  IdealPFdbkVariant=Disabled  SatFdbkVariant=Disabled  DerivativeFilterVariant=Disabled  NVariant=Disabled  NCopyVariant=Disabled_SignalSpec  FilterICVariant=Disabled  IntegratorICVariant=InternalICs  ExternalResetVariant=Disabled  TRSumVariant=Passthrough  SumFdbkVariant=Disabled  SumVariant=Sum_PI  TsampFilterVariant=InternalTs  TsampNgainVariant=Passthrough  TsampIntegralVariant=Disabled_SignalSpec  ExternalSaturationOutDataTypeStr=Inherit: Same as second input  DerivativeSourceVariant=Disabled  PreIntVariant=InternalPreInt
  vc : Outport
  wires:
  PI Controller/1 -> vc/1
  error/1 -> PI Controller/1

== system ConverterLibrary/Controller/Power Factor Correction Converters/Interleaved Boost PFC Controller/Current Balance/Balance Controller/PIDiscrete ==
  error : Inport
  PI Controller : slpidlib/PID Controller  Controller=PI  Form=Parallel  TimeDomain=Discrete-time  UseExternalTs=off  SampleTime=TsCurrent  IntegratorMethod=Backward Euler  FilterMethod=Forward Euler  ControllerParametersSource=internal  P=KpBalance  I=KiBalance  UseKiTs=off  D=0  UseExternalDerivativeSource=off  N=100  UseFilter=on  TunerSelectOption=Transfer Function Based (PID Tuner App)  InitialConditionSource=internal  InitialConditionForIntegrator=0  InitialConditionForFilter=0  DifferentiatorICPrevScaledInput=0  ExternalReset=none  TrackingMode=off  Kt=1  LimitOutput=on  SatLimitsSource=internal  UpperSaturationLimit=dutyBalanceMax  LowerSaturationLimit=-dutyBalanceMax  LinearizeAsGain=on  AntiWindupMode=clamping  Kb=1  LimitIntegrator=on  UpperIntegratorSaturationLimit=dutyBalanceMax  LowerIntegratorSaturationLimit=-dutyBalanceMax  POutMin=[]  POutMax=[]  IOutMin=[]  IOutMax=[]  DOutMin=[]  DOutMax=[]  NOutMin=[]  NOutMax=[]  SumOutMin=[]  SumOutMax=[]  SaturationOutMin=[]  SaturationOutMax=[]  PParamMin=[]  PParamMax=[]  IParamMin=[]  IParamMax=[]  DParamMin=[]  DParamMax=[]  NParamMin=[]  NParamMax=[]  KbParamMin=[]  KbParamMax=[]  KtParamMin=[]  KtParamMax=[]  KbOutMin=[]  KbOutMax=[]  KtOutMin=[]  KtOutMax=[]  IntegratorOutMin=[]  IntegratorOutMax=[]  FilterOutMin=[]  FilterOutMax=[]  SumI1OutMin=[]  SumI1OutMax=[]  SumI2OutMin=[]  SumI2OutMax=[]  SumI3OutMin=[]  SumI3OutMax=[]  SumI4OutMin=[]  SumI4OutMax=[]  SumDOutMin=[]  SumDOutMax=[]  DifferentiatorOutMin=[]  DifferentiatorOutMax=[]  FilterDiffOutCoefMin=[]  FilterDiffOutCoefMax=[]  ReciprocalOutMin=[]  ReciprocalOutMax=[]  SumDenOutMin=[]  SumDenOutMax=[]  SumNumOutMin=[]  SumNumOutMax=[]  DivideOutMin=[]  DivideOutMax=[]  UdiffTsProdOutMin=[]  UdiffTsProdOutMax=[]  NTsProdOutMin=[]  NTsProdOutMax=[]  UintegralTsProdOutMin=[]  UintegralTsProdOutMax=[]  UngainTsProdOutMin=[]  UngainTsProdOutMax=[]  ClampingZeroOutDataTypeStr=Inherit: Inherit via back propagation  ClampingZeroOutMin=[]  ClampingZeroOutMax=[]  FilterDenConstantOutDataTypeStr=Inherit: Inherit via back propagation  FilterDenConstantOutMin=[]  FilterDenConstantOutMax=[]  PCopyOutDataTypeStr=Inherit: Inherit via back propagation  PCopyOutMin=[]  PCopyOutMax=[]  NCopyOutDataTypeStr=Inherit: Inherit via back propagation  NCopyOutMin=[]  NCopyOutMax=[]  IntegratorContinuousStateAttributes=''  IntegratorStateMustResolveToSignalObject=off  IntegratorRTWStateStorageClass=Auto  FilterContinuousStateAttributes=''  FilterStateMustResolveToSignalObject=off  FilterRTWStateStorageClass=Auto  ParallelPVariant=InternalParameters  IdealPVariant=Disabled  IVariant=InternalParameters  DVariant=Disabled  IntegratorVariant=Discrete  SatVariant=Enabled  AWVariant=DiscClampingParallel  PCopyVariant=Disabled  TRVariant=Disabled  FdbkBlocksVariant=Feedback  IdealPFdbkVariant=Passthrough  SatFdbkVariant=Passthrough  DerivativeFilterVariant=Disabled  NVariant=Disabled  NCopyVariant=Disabled_SignalSpec  FilterICVariant=Disabled  IntegratorICVariant=InternalICs  ExternalResetVariant=Disabled  TRSumVariant=Passthrough  SumFdbkVariant=Enabled  SumVariant=Sum_PI  TsampFilterVariant=InternalTs  TsampNgainVariant=Passthrough  TsampIntegralVariant=Disabled_SignalSpec  ExternalSaturationOutDataTypeStr=Inherit: Same as second input  DerivativeSourceVariant=Disabled  PreIntVariant=InternalPreInt
  vc : Outport
  wires:
  PI Controller/1 -> vc/1
  error/1 -> PI Controller/1

== system ConverterLibrary/Controller/Power Factor Correction Converters/Interleaved Boost PFC Controller/Output Mode/PWMSignal/Gate Drive ==
  gateLogic : Inport
  Gate Level Span : Gain  Gain=gateVoltageOn - gateVoltageOff
  Gate Off Level : Bias  Bias=gateVoltageOff  SaturateOnIntegerOverflow=off
  gateVoltage : Outport
  wires:
  Gate Off Level/1 -> gateVoltage/1
  Gate Level Span/1 -> Gate Off Level/1
  gateLogic/1 -> Gate Level Span/1

== system ConverterLibrary/Controller/Power Factor Correction Converters/Interleaved Boost PFC Controller/Output Mode/PWMSignal/Leg Gate Logic ==
  Ton : Inport
  Toff : Inport  Port=2
  S : Inport  Port=3
  After Turn Off : RelationalOperator
  After Turn On : RelationalOperator
  Pulse Window : Logic  Operator=XOR
  To Double : DataTypeConversion  OutDataTypeStr=double
  gates : Outport
  wires:
  Ton/1 -> After Turn On/2
  Toff/1 -> After Turn Off/2
  S/1 -> After Turn Off/1, After Turn On/1
  After Turn On/1 -> Pulse Window/1
  After Turn Off/1 -> Pulse Window/2
  Pulse Window/1 -> To Double/1
  To Double/1 -> gates/1

== system ConverterLibrary/Controller/Power Factor Correction Converters/Interleaved Boost PFC Controller/Output Mode/PWMSignal/Ramp Mode ==
  Tsw : Inport
  FixedStep : Subsystem  VariantControl=FixedStep
  VariableStep : Subsystem  VariantControl=VariableStep
  S : Outport

== system ConverterLibrary/Controller/Power Factor Correction Converters/Totem-Pole Boost PFC Controller/Gate Logic/Slow Leg Complementary PWM/Convert2Double ==
  In1 : Inport
  Logic To Double : DataTypeConversion  OutDataTypeStr=double
  Rate Offset : Bias  Bias=-1
  Rate Swing : Gain  Gain=2
  Out1 : Outport
  wires:
  Logic To Double/1 -> Rate Swing/1
  Rate Swing/1 -> Rate Offset/1
  Rate Offset/1 -> Out1/1
  In1/1 -> Logic To Double/1

== system ConverterLibrary/Controller/Power Factor Correction Converters/Totem-Pole Boost PFC Controller/Gate Logic/Slow Leg Complementary PWM/GateVoltage ==
  in : Inport
  Gate Level Offset : Bias  Bias=gateVoltageOff
  Gate Level Swing : Gain  Gain=gateVoltageOn - gateVoltageOff
  To Double : DataTypeConversion  OutDataTypeStr=double
  G : Outport
  wires:
  Gate Level Swing/1 -> Gate Level Offset/1
  To Double/1 -> Gate Level Swing/1
  Gate Level Offset/1 -> G/1
  in/1 -> To Double/1

== system ConverterLibrary/Controller/Power Factor Correction Converters/Totem-Pole Boost PFC Controller/Gate Logic/Slow Leg Complementary PWM/Ramp Mode ==
  rate : Inport
  FixedStep : Subsystem  VariantControl=FixedStep
  VariableStep : Subsystem  VariantControl=VariableStep
  S : Outport

== system ConverterLibrary/Controller/Power Factor Correction Converters/Totem-Pole Boost PFC Controller/Output Mode/PWMSignal/Half Bridge PWM Generator ==
  duty : Inport
  Dead Time : Constant  Value=(fastLegDeadTime)
  Gate Level Offset : Bias  Bias=gateVoltageOff
  Gate Level Swing : Gain  Gain=gateVoltageOn - gateVoltageOff
  Leg Gate Logic : Subsystem
  Pulse Time : Gain  Gain=1/Fsw
  Pulse Time Plus Dead Time : Bias  Bias=(fastLegDeadTime)
  Pulse Width Limit : Saturate  UpperLimit=1 - (fastLegDeadTime)*Fsw  LowerLimit=(fastLegDeadTime)*Fsw
  Ramp Mode : Subsystem  Variant=on  VariantControlMode=label  LabelModeActiveChoice=VariableStep
  Switching Period : Constant  Value=1/Fsw
  Turn Off Times : Mux  Inputs=2
  Turn On Times : Mux  Inputs=2
  G : Outport
  wires:
  Gate Level Offset/1 -> G/1
  Leg Gate Logic/1(gates) -> Gate Level Swing/1
  Ramp Mode/1(S) -> Leg Gate Logic/3(S)
  Turn Off Times/1 -> Leg Gate Logic/2(Toff)
  Turn On Times/1 -> Leg Gate Logic/1(Ton)
  Gate Level Swing/1 -> Gate Level Offset/1
  Switching Period/1 -> Ramp Mode/1(Tsw), Turn Off Times/2
  Pulse Time Plus Dead Time/1 -> Turn On Times/2
  Dead Time/1 -> Turn On Times/1
  Pulse Time/1 -> Turn Off Times/1, Pulse Time Plus Dead Time/1
  Pulse Width Limit/1 -> Pulse Time/1
  duty/1 -> Pulse Width Limit/1

== system ConverterLibrary/Controller/Soft-Switching Converters/CLLC Controller/Gate Signal/CLLC PWM Generator/Primary Gate Signal ==
  fpu : Inport
  Bridge Gate Map : Selector  InputPortWidth=2  IndexOptions=Index vector (dialog)  Indices=[1 2 2 1]  OutputSizes=1
  Dead Time : Constant  Value=Tdead
  Gate Level Offset : Bias  Bias=(0)
  Gate Level Swing : Gain  Gain=(10) - (0)
  Hertz To Period : Math  Operator=reciprocal
  Leg Gate Logic : Subsystem
  Normalized To Hertz : Gain  Gain=(resFreq)
  Primary Gates To Logic : DataTypeConversion  OutDataTypeStr=boolean
  Pulse Time : Gain  Gain=(0.5)
  Pulse Time Plus Dead Time : Bias  Bias=Tdead
  Ramp Mode : Subsystem  Variant=on  VariantControlMode=label  LabelModeActiveChoice=VariableStep
  Turn Off Times : Mux  Inputs=2
  Turn On Times : Mux  Inputs=2
  G : Outport
  gates : Outport  Port=2
  wires:
  Gate Level Swing/1 -> Gate Level Offset/1
  fpu/1 -> Normalized To Hertz/1
  Normalized To Hertz/1 -> Hertz To Period/1
  Hertz To Period/1 -> Pulse Time/1, Turn Off Times/2, Ramp Mode/1(Tsw)
  Pulse Time/1 -> Pulse Time Plus Dead Time/1, Turn Off Times/1
  Dead Time/1 -> Turn On Times/1
  Pulse Time Plus Dead Time/1 -> Turn On Times/2
  Turn On Times/1 -> Leg Gate Logic/1(Ton)
  Turn Off Times/1 -> Leg Gate Logic/2(Toff)
  Ramp Mode/1(S) -> Leg Gate Logic/3(S)
  Leg Gate Logic/1(gates) -> Bridge Gate Map/1
  Bridge Gate Map/1 -> Gate Level Swing/1, Primary Gates To Logic/1
  Gate Level Offset/1 -> G/1
  Primary Gates To Logic/1 -> gates/1

== system ConverterLibrary/Controller/Soft-Switching Converters/CLLC Controller/Gate Signal/CLLC PWM Generator/Synchronous Rectifier ==
  primaryGates : Inport
  fpu : Inport  Port=2
  Isec : Inport  Port=3
  Conduction Detect : Subsystem
  Rectifier Gate Level Offset : Bias  Bias=(0)
  Rectifier Gate Level Swing : Gain  Gain=(10) - (0)
  Rectifier Gates To Double : DataTypeConversion  OutDataTypeStr=double
  Region Select : Subsystem
  Turn On Delay : Subsystem
  Gs : Outport
  wires:
  Rectifier Gate Level Swing/1 -> Rectifier Gate Level Offset/1
  primaryGates/1 -> Region Select/1(primaryGates)
  fpu/1 -> Region Select/2(fpu)
  Isec/1 -> Conduction Detect/1(Isec)
  Conduction Detect/1(permit) -> Region Select/3(permit)
  Region Select/1(Gs) -> Turn On Delay/1(condition)
  Turn On Delay/1(Gs) -> Rectifier Gates To Double/1
  Rectifier Gates To Double/1 -> Rectifier Gate Level Swing/1
  Rectifier Gate Level Offset/1 -> Gs/1

== system ConverterLibrary/Controller/Soft-Switching Converters/CLLC Controller/VCO/TwoRate/If Action Subsystem ==
  In1 : Inport
  Action Port : ActionPort
  Gain : Gain  Gain=vcoGainVec(2)
  Out1 : Outport
  wires:
  Gain/1 -> Out1/1
  In1/1 -> Gain/1

== system ConverterLibrary/Controller/Soft-Switching Converters/CLLC Controller/VCO/TwoRate/If Action Subsystem1 ==
  In1 : Inport
  Action Port : ActionPort
  Gain : Gain  Gain=vcoGainVec(1)
  Out1 : Outport
  wires:
  Gain/1 -> Out1/1
  In1/1 -> Gain/1

== system ConverterLibrary/Controller/Soft-Switching Converters/CLLC Controller/Voltage Controller/If Action Subsystem1/Voltage PI ==
  note: 1) Add Subsystem or Model blocks as valid variant choices.
      | 2) You cannot connect blocks at this level. At simulation, connectivity is automatically
      | determined, based on the active variant and port name matching.
  error : Inport
  PIContinuous : Subsystem  VariantControl=PIContinuous
  PIDiscrete : Subsystem  VariantControl=PIDiscrete
  vc : Outport

== system ConverterLibrary/Controller/Soft-Switching Converters/DAB Controller (SPS)/CC-CV Control/CC Mode/Controller ==
  error : Inport
  PIContinuous : Subsystem  VariantControl=PIContinuous
  PIDiscrete : Subsystem  VariantControl=PIDiscrete
  vc : Outport

== system ConverterLibrary/Controller/Soft-Switching Converters/DAB Controller (SPS)/CC-CV Control/CV Mode/Voltage PI ==
  error : Inport
  PIContinuous : Subsystem  VariantControl=PIContinuous
  PIDiscrete : Subsystem  VariantControl=PIDiscrete
  vc : Outport
